simulink model "SZ04_ARM"  (R2026a)
settings: Solver=VariableStepAuto  MaxStep=tau/25
InitFcn:
  | K = 5;
  | tau = 0.125;
  | 
  | y_0 = 2.5;
settings Model: Creator=Szalay  LastModifiedBy=Szalay

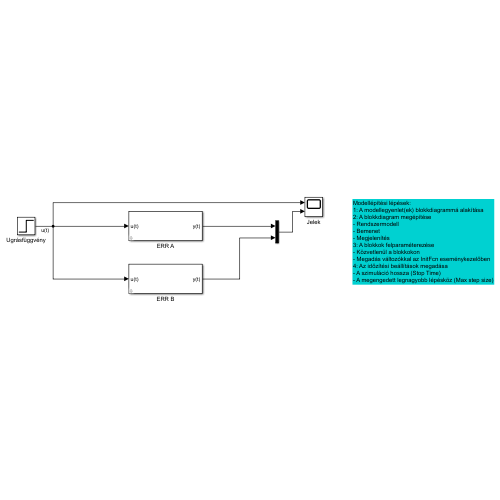
[thumbnail: Simulink's stored preview of the top-level diagram]
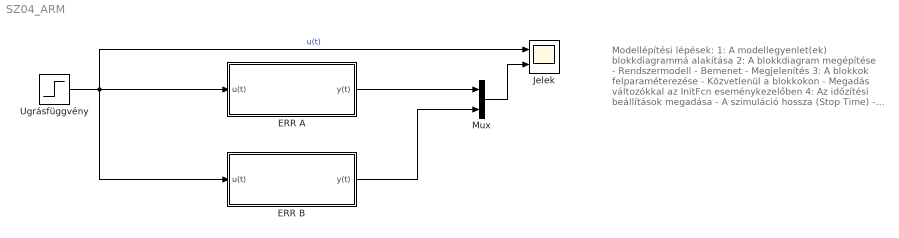
== system SZ04_ARM ==
  note: Modellépítési lépések:
      | 1: A modellegyenlet(ek) blokkdiagrammá alakítása
      | 2: A blokkdiagram megépítése
      | - Rendszermodell
      | - Bemenet
      | - Megjelenítés
      | 3: A blokkok felparaméterezése
      | - Közvetlenül a blokkokon
      | - Megadás változókkal az InitFcn eseménykezelőben
      | 4: Az időzítési beállítások megadása
      | - A szimuláció hossza (Stop Time)
      | - A megengedett legnagyobb lépésköz (Max step size)
  ERR A : Subsystem  mask(Elsőrendű rendszer){K=1, tau=1, y_0=0}
      mask prompts: K "Állandósult állapoti erősítés"; tau "Időállandó"; y_0 "A kimenet kezdeti értéke"
      mask help: A lineáris elsőrendű rendszer modellje.
      mask DialogControl ParameterGroupVar Prompt: Rendszerparaméterek
      mask DialogControl Container3 Prompt: Kezdeti érték
  ERR B : Subsystem  mask(Elsőrendű rendszer){K=2, tau=1, y_0=2}
      mask prompts: K "Állandósult állapoti erősítés"; tau "Időállandó"; y_0 "A kimenet kezdeti értéke"
      mask help: A lineáris elsőrendű rendszer modellje.
      mask DialogControl ParameterGroupVar Prompt: Rendszerparaméterek
      mask DialogControl Container3 Prompt: Kezdeti érték
  Jelek : Scope  NumInputPorts=2
      settings: ActiveDisplayYMinimum=-0.31249999999999994  ActiveDisplayYMaximum=2.8125
  Mux : Mux  Inputs=2
  Ugrásfüggvény : Step  Time=5  SampleTime=0
  wires:
  Ugrásfüggvény/1 -> ERR B/1(u(t)), Jelek/1, ERR A/1(u(t))  "u(t)"
  Mux/1 -> Jelek/2
  ERR A/1(y(t)) -> Mux/1
  ERR B/1(y(t)) -> Mux/2

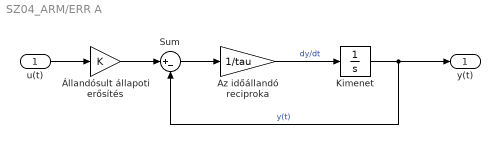
== system SZ04_ARM/ERR A ==
  u(t) : Inport
  Az időállandó reciproka : Gain  Gain=1/tau
  Kimenet : Integrator  InitialCondition=y_0
  Sum : Sum  Inputs=|+-
  Állandósult állapoti erősítés : Gain  Gain=K
  y(t) : Outport
  wires:
  Kimenet/1 -> y(t)/1, Sum/2  "y(t)"
  Az időállandó reciproka/1 -> Kimenet/1  "dy/dt"
  Állandósult állapoti erősítés/1 -> Sum/1
  Sum/1 -> Az időállandó reciproka/1
  u(t)/1 -> Állandósult állapoti erősítés/1

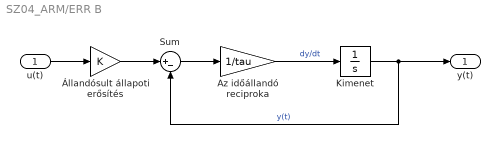
== system SZ04_ARM/ERR B ==
  u(t) : Inport
  Az időállandó reciproka : Gain  Gain=1/tau
  Kimenet : Integrator  InitialCondition=y_0
  Sum : Sum  Inputs=|+-
  Állandósult állapoti erősítés : Gain  Gain=K
  y(t) : Outport
  wires:
  u(t)/1 -> Állandósult állapoti erősítés/1
  Sum/1 -> Az időállandó reciproka/1
  Állandósult állapoti erősítés/1 -> Sum/1
  Az időállandó reciproka/1 -> Kimenet/1  "dy/dt"
  Kimenet/1 -> Sum/2, y(t)/1  "y(t)"
